simulink model "ASM_Traffic_MultiCore"  (R2026a)
settings: Solver=ode1  StartTime=SIM.tstart.v  StopTime=SIM.tend.v  FixedStep=SIM.StepSize.v
PostLoadFcn:
  | if any(exist('dsrtsu_mdlpostloadfcn', 'file') ~= 0), dsrtsu_mdlpostloadfcn('Execute', bdroot); end
  | try, asm_mdl_postloadfcn(bdroot, 'UpdateModel', 3600); catch, disp(lasterr); end,
InitFcn:
  | , if any(exist('rtifpga_mdlclblib', 'file') ~= 0), rtifpga_mdlclblib('Init', bdroot); end,
  | , if any(exist('dsmpb_private', 'file') ~= 0), dsmpb_private('dsmpb_mdlclblib', 'Init', bdroot); end,
model workspace (MAT data in the model file):
  asmReferencePath = [0 0.01 0.02 0.03 0.04 0.05 0.06 0.07 0.08 0.09 0.1 0.11 ... (350007 elements, 50001x7)]
  roadBounds : Simulink.Parameter (value not decoded)
  safetyAxes : Simulink.Parameter (value not decoded)
undefined symbols (not defined in the file): _to_, a0b2, ASM_BrakeHydraulics_DemoSystems, ASM_VehicleDynamics_DemoSystems, b98103fe8ad365046cd0, BrakeCircuit, controllerConfig, CPT, Crankshaft, DiscIntNeverNeededParam, dsmsi, FinalDriveAssembly, MDL, ModeSignals, mu, Pos_BrakePedal_Maneuver, rad, RefSignals, roadFamilyData, roadFamilyId, s_to_rpm, SIM, SoftECU, Suspension, Tire, Transmission
libraries: ASM_Traffic_lib x135, simulink x98, ASM_Utils_lib x77, ASM_VehicleDynamics_lib x70, ASM_Environment_lib x22, dsmpblib x20, dsmsilib x15, MDLD_Utils_lib x10, ASM_BrakeHydraulics_lib x3, sl_discontinuities x2
(part 37 of 65)

== system ASM_Traffic_MultiCore/Driver/Plant/Driver/ReferenceVelocity/Reduce_Dimension2 ==
  In : Inport
  Selector : Selector  InputPortWidth=15  IndexOptions=Index vector (dialog)  Indices=[8:10]  OutputSizes=1
      settings: AttributesFormatString=|
      | PortWidth = %<InputPortWidth>
      | Indices = %<Indices>
  UnitConversion2 : ASM_Utils_lib/UnitConversion/UnitConversion  Selection=km/h_to_m/s
  Out : Outport  VectorParamsAs1DForOutWhenUnconnected=off
  wires:
  UnitConversion2/1 -> Selector/1
  In/1 -> UnitConversion2/1
  Selector/1 -> Out/1

== system ASM_Traffic_MultiCore/Driver/Plant/Driver/ReferenceVelocity/Reduce_Dimension3 ==
  In : Inport
  Selector : Selector  InputPortWidth=15  IndexOptions=Index vector (dialog)  Indices=[1:10]  OutputSizes=1
      settings: AttributesFormatString=|
      | PortWidth = %<InputPortWidth>
      | Indices = %<Indices>
  Out : Outport  VectorParamsAs1DForOutWhenUnconnected=off
  wires:
  In/1 -> Selector/1
  Selector/1 -> Out/1

== system ASM_Traffic_MultiCore/Driver/Plant/Driver/ReferenceVelocity/Reduce_Dimension4 ==
  In : Inport
  Selector : Selector  InputPortWidth=10  IndexOptions=Index vector (dialog)  Indices=[8:10]  OutputSizes=1
      settings: AttributesFormatString=|
      | PortWidth = %<InputPortWidth>
      | Indices = %<Indices>
  Out : Outport  VectorParamsAs1DForOutWhenUnconnected=off
  wires:
  Selector/1 -> Out/1
  In/1 -> Selector/1

== system ASM_Traffic_MultiCore/Driver/Plant/UserInterface/DISP_Plant/Angle_SteeringWheel[deg] ==
  In1 : Inport
  Out1 : Outport  VectorParamsAs1DForOutWhenUnconnected=off
  wires:
  In1/1 -> Out1/1

== system ASM_Traffic_MultiCore/Driver/Plant/UserInterface/DISP_Plant/Err ==
  Current : Inport
  Set : Inport  Port=2
  Sum : Sum  Inputs=|+-  InputSameDT=on  SaturateOnIntegerOverflow=on  OutDataTypeStr=Inherit: Same as first input
  Error[km|h] : Outport  VectorParamsAs1DForOutWhenUnconnected=off
  wires:
  Current/1 -> Sum/1
  Set/1 -> Sum/2
  Sum/1 -> Error[km|h]/1

== system ASM_Traffic_MultiCore/Driver/Plant/UserInterface/DISP_Plant/Gear[] ==
  In1 : Inport
  Out1 : Outport  VectorParamsAs1DForOutWhenUnconnected=off
  wires:
  In1/1 -> Out1/1

== system ASM_Traffic_MultiCore/Driver/Plant/UserInterface/DISP_Plant/Pos_AccPedal[%] ==
  In1 : Inport
  Out1 : Outport  VectorParamsAs1DForOutWhenUnconnected=off
  wires:
  In1/1 -> Out1/1

== system ASM_Traffic_MultiCore/Driver/Plant/UserInterface/DISP_Plant/Pos_BrakePedal[%] ==
  In1 : Inport
  Out1 : Outport  VectorParamsAs1DForOutWhenUnconnected=off
  wires:
  In1/1 -> Out1/1

== system ASM_Traffic_MultiCore/Driver/Plant/UserInterface/DISP_Plant/Pos_ClutchPedal[%] ==
  In1 : Inport
  Out1 : Outport  VectorParamsAs1DForOutWhenUnconnected=off
  wires:
  In1/1 -> Out1/1

== system ASM_Traffic_MultiCore/Driver/Plant/UserInterface/DISP_Plant/RelativeErr ==
  Current : Inport
  Set : Inport  Port=2
  AvoidNAN : Fcn  Expr=u/(u*u+1.E-20)
  Limit_RelativeError : Saturate  UpperLimit=UpLim  LowerLimit=LowLim
  Product : Product  InputSameDT=on  SaturateOnIntegerOverflow=on  OutDataTypeStr=Inherit: Same as first input
  Sum : Sum  Inputs=|+-  InputSameDT=on  SaturateOnIntegerOverflow=on  OutDataTypeStr=Inherit: Same as first input
  "[0_1]2[%]" : Gain  Gain=100  SaturateOnIntegerOverflow=on  OutDataTypeStr=Inherit: Same as input  ParamDataTypeStr=Inherit: Same as input
  RelativeError[%] : Outport  VectorParamsAs1DForOutWhenUnconnected=off
  wires:
  AvoidNAN/1 -> Product/2
  Current/1 -> Sum/1
  Product/1 -> "[0_1]2[%]"/1
  Set/1 -> AvoidNAN/1, Sum/2
  Sum/1 -> Product/1
  "[0_1]2[%]"/1 -> Limit_RelativeError/1
  Limit_RelativeError/1 -> RelativeError[%]/1

== system ASM_Traffic_MultiCore/Driver/Plant/UserInterface/DISP_Plant/SelectorLever[-3T|-2P|-1R|0N|1D] ==
  In1 : Inport
  Out1 : Outport  VectorParamsAs1DForOutWhenUnconnected=off
  wires:
  In1/1 -> Out1/1

== system ASM_Traffic_MultiCore/Driver/Plant/UserInterface/DISP_Plant/a_x_Vehicle_Ref[m|s2] ==
  In1 : Inport
  Out1 : Outport  VectorParamsAs1DForOutWhenUnconnected=off
  wires:
  In1/1 -> Out1/1

== system ASM_Traffic_MultiCore/Driver/Plant/UserInterface/DISP_Plant/e_Lat[m] ==
  In1 : Inport
  Out1 : Outport  VectorParamsAs1DForOutWhenUnconnected=off
  wires:
  In1/1 -> Out1/1

== system ASM_Traffic_MultiCore/Driver/Plant/UserInterface/DISP_Plant/v_Vehicle[km|h] ==
  In1 : Inport
  Out1 : Outport  VectorParamsAs1DForOutWhenUnconnected=off
  wires:
  In1/1 -> Out1/1

== system ASM_Traffic_MultiCore/Driver/Plant/UserInterface/DISP_Plant/v_Vehicle_Ref[km|h] ==
  In1 : Inport
  Out1 : Outport  VectorParamsAs1DForOutWhenUnconnected=off
  wires:
  In1/1 -> Out1/1

== system ASM_Traffic_MultiCore/Driver/SignalInterface/ASMSignalInterface/signal_structure/InfoBlock ==

== system ASM_Traffic_MultiCore/Drivetrain/Control/SoftECU_Drivetrain/SoftECU_Transmission/ASMSignalCollector ==
  BusCreator : BusCreator  Inputs=5
  ASMSignalBus : Outport  VectorParamsAs1DForOutWhenUnconnected=off
  wires:
  BusCreator/1 -> ASMSignalBus/1  "Control"
  [ASMBUS_SOFTECU_LOCKUP_CLUTCH_CONTROL] -> BusCreator/1
  [ASMBUS_SOFTECU_SHIFT_LOCK_CONTROL] -> BusCreator/2
  [ASMBUS_SOFTECU_SHIFT_STRATEGY] -> BusCreator/3
  [ASMBUS_SOFTECU_TIP_SHIFT_CONTROL] -> BusCreator/4
  [ASMBUS_SOFTECU_TORQUE_INTERVENTION_CONTROL] -> BusCreator/5

== system ASM_Traffic_MultiCore/Drivetrain/Control/SoftECU_Drivetrain/SoftECU_Transmission/SOFTECU_SETUP ==
  Gear_Max_Maneuver[0Off|1_n] : Inport
  SOFTECU_TRANSMISSION_SETUP : ASM_VehicleDynamics_lib/SoftECU/SoftECU_Transmission/SOFTECU_TRANSMISSION_SETUP  Tag=ASM_SUBCOMPONENT  Const_Max_num_Gear=MDL.SoftECU.SoftECUTransmission.Const_Max_num_Gear  ASMProperties=struct('Name','SOFTECU_TRANSMISSION_SETUP','Version','1.0','Library','ASM_VehicleDynamics_lib')  ASMInstanceName=softecu_transmission_setup  ASMInstanceID=1
  Terminator : Terminator
  tag scope: TAG_SoftECU_Const_Max_num_Gear=scoped
  wires:
  SOFTECU_TRANSMISSION_SETUP/1 -> [TAG_SoftECU_Const_Max_num_Gear]
  [TAG_SoftECU_Const_Max_num_Gear] -> Terminator/1
  Gear_Max_Maneuver[0Off|1_n]/1 -> SOFTECU_TRANSMISSION_SETUP/1

== system ASM_Traffic_MultiCore/Drivetrain/Control/SoftECU_Drivetrain/SoftECU_Transmission/State_Engine ==
  note: Consider the engine to be active, if StartStop system is active
  In[] : Inport
  State_StartStop[1Off|2NotReady|3Ready|4EngStopped] : Inport  Port=2
  Data Type Conversion : DataTypeConversion  OutDataTypeStr=double  SaturateOnIntegerOverflow=off  RndMeth=Floor
  Engine_Active : Constant  Value=3
  NotOff : simulink/Logic and Bit Operations/Compare To Constant  relop=~=  const=1  OutDataTypeStr=boolean
  Switch : Switch  Criteria=u2 ~= 0  SaturateOnIntegerOverflow=off  InputSameDT=off
  Out[] : Outport  VectorParamsAs1DForOutWhenUnconnected=off
  wires:
  State_StartStop[1Off|2NotReady|3Ready|4EngStopped]/1 -> NotOff/1
  Data Type Conversion/1 -> Switch/3
  NotOff/1 -> Switch/2
  Switch/1 -> Out[]/1
  Engine_Active/1 -> Switch/1
  In[]/1 -> Data Type Conversion/1

== system ASM_Traffic_MultiCore/Drivetrain/Control/SoftECU_Drivetrain/SoftECU_Transmission/Sw_Gear ==
  In[] : Inport
  Ext : Constant
  OR : Logic  Operator=OR  AllPortsSameDT=off  OutDataTypeStr=boolean
  Ref : simulink/Logic and Bit Operations/Compare To Constant  relop===  const=4  OutDataTypeStr=boolean
  SoftECU : Constant  Value=2
  Stim : simulink/Logic and Bit Operations/Compare To Constant  relop===  const=1  OutDataTypeStr=boolean
  Switch : Switch  Criteria=u2 ~= 0  SaturateOnIntegerOverflow=off  InputSameDT=off
  Terminator : Terminator
  Out[] : Outport  VectorParamsAs1DForOutWhenUnconnected=off
  wires:
  Switch/1 -> Terminator/1
  SoftECU/1 -> Switch/3, Out[]/1
  Ext/1 -> Switch/1
  OR/1 -> Switch/2
  Ref/1 -> OR/2
  Stim/1 -> OR/1
  In[]/1 -> Ref/1, Stim/1

== system ASM_Traffic_MultiCore/Drivetrain/Control/SoftECU_Drivetrain/SoftECU_Transmission/Sw_LockupClutch ==
  In[] : Inport
  SoftECU : Constant  Value=2
  Terminator : Terminator
  Out[] : Outport  VectorParamsAs1DForOutWhenUnconnected=off
  wires:
  SoftECU/1 -> Out[]/1
  In[]/1 -> Terminator/1

== system ASM_Traffic_MultiCore/Drivetrain/Control/SoftECU_Drivetrain/SoftECU_Transmission/Unit Delay ==
  In1 : Inport
  Reset_States[0|1] : Inport  Port=2
  Unit Delay Resettable1 : Delay  DelayLength=1  InitialCondition=0  ExternalReset=Level
      settings: InputPortMap=u0,r5
  Out1 : Outport  VectorParamsAs1DForOutWhenUnconnected=off
  wires:
  Reset_States[0|1]/1 -> Unit Delay Resettable1/2
  In1/1 -> Unit Delay Resettable1/1
  Unit Delay Resettable1/1 -> Out1/1

== system ASM_Traffic_MultiCore/Drivetrain/Control/SoftECU_Drivetrain/SoftECU_Transmission/Unit Delay2 ==
  In1 : Inport
  Reset_States[0|1] : Inport  Port=2
  Unit Delay Resettable1 : Delay  DelayLength=1  InitialCondition=100  ExternalReset=Level
      settings: InputPortMap=u0,r5
  Out1 : Outport  VectorParamsAs1DForOutWhenUnconnected=off
  wires:
  Reset_States[0|1]/1 -> Unit Delay Resettable1/2
  In1/1 -> Unit Delay Resettable1/1
  Unit Delay Resettable1/1 -> Out1/1

== system ASM_Traffic_MultiCore/Drivetrain/Control/UserInterface/DISP_Control/Ctrl_Lockup_Clutch[0_1] ==
  In1 : Inport
  Out1 : Outport  VectorParamsAs1DForOutWhenUnconnected=off
  wires:
  In1/1 -> Out1/1

== system ASM_Traffic_MultiCore/Drivetrain/Control/UserInterface/DISP_Control/Ctrl_Parking_Pawl[0|1] ==
  In1 : Inport
  Out1 : Outport  VectorParamsAs1DForOutWhenUnconnected=off
  wires:
  In1/1 -> Out1/1

== system ASM_Traffic_MultiCore/Drivetrain/Control/UserInterface/DISP_Control/Factor_Trq_Engine_Red[%] ==
  In1 : Inport
  Out1 : Outport  VectorParamsAs1DForOutWhenUnconnected=off
  wires:
  In1/1 -> Out1/1

== system ASM_Traffic_MultiCore/Drivetrain/Control/UserInterface/DISP_Control/Gear[] ==
  In1 : Inport
  Out1 : Outport  VectorParamsAs1DForOutWhenUnconnected=off
  wires:
  In1/1 -> Out1/1

== system ASM_Traffic_MultiCore/Drivetrain/Plant/Drivetrain/Final_Drive_Assembly/ASMSignalCollector ==
  Bus Selector1 : BusSelector  OutputSignals=Shaft_FL,Shaft_FR
  Bus Selector2 : BusSelector  OutputSignals=Shaft_RL,Shaft_RR
  BusCreator : BusCreator  Inputs=18
  Clutch_4WD : Subsystem
  Dummy_TGCL4WD_Shaft : Subsystem
  FinalDriveRatio : Subsystem
  Shaft_CF : Subsystem
  Shaft_CR : Subsystem
  Transfer_Gearbox : Subsystem
  Trq_Shafts : Subsystem
  tag scope: ASMBUS_Drivetrain_FinalDriveAssembly=scoped
  wires:
  Trq_Shafts/2(Trq_Shaft[FL;FR;RL;RR][Nm]) -> BusCreator/18
  Trq_Shafts/1(Trq_Out_Front_Diff[Nm]) -> BusCreator/17
  FinalDriveRatio/4(i_FinalDrive[]) -> BusCreator/4
  FinalDriveRatio/3(TrqDistri_Front_Rear[0_1]) -> BusCreator/3
  FinalDriveRatio/2(i_RearDrive[]) -> BusCreator/2
  FinalDriveRatio/1(i_FrontDrive[]) -> BusCreator/1
  BusCreator/1 -> [ASMBUS_Drivetrain_FinalDriveAssembly]  "FinalDriveAssembly"
  Bus Selector2/2 -> BusCreator/16, Trq_Shafts/4(Shaft_RR)  "<Shaft_RR>"
  Bus Selector2/1 -> BusCreator/15, Trq_Shafts/3(Shaft_RL)  "<Shaft_RL>"
  Bus Selector1/2 -> BusCreator/14, Trq_Shafts/2(Shaft_FR)  "<Shaft_FR>"
  Bus Selector1/1 -> BusCreator/13, Trq_Shafts/1(Shaft_FL)  "<Shaft_FL>"
  Clutch_4WD/1(ASMSignalBus) -> BusCreator/12
  Transfer_Gearbox/1(ASMSignalBus) -> BusCreator/11
  [ASMBUS_Drivetrain_CentralDifferential] -> FinalDriveRatio/2(CentralDifferential), BusCreator/5
  Dummy_TGCL4WD_Shaft/1(Out) -> BusCreator/8
  [ASMBUS_Drivetrain_RearDifferential] -> BusCreator/7, FinalDriveRatio/4(RearDifferential), Bus Selector2/1
  [ASMBUS_Drivetrain_FrontDifferential] -> BusCreator/6, FinalDriveRatio/3(FrontDifferential), Bus Selector1/1
  Shaft_CF/1(ASMSignalBus) -> BusCreator/9
  Shaft_CR/1(ASMSignalBus) -> BusCreator/10
  [ASMBUS_Drivetrain_Mode] -> Shaft_CF/1(Mode_Drivetrain[1|2|3|4|5]), Clutch_4WD/1(Mode_Drivetrain[1|2|3|4|5]), Transfer_Gearbox/1(Mode_Drivetrain[1|2|3|4|5]), Shaft_CR/1(Mode_Drivetrain[1|2|3|4|5]), FinalDriveRatio/1(Drivetrain_Mode[1|2|3|4|5])

== system ASM_Traffic_MultiCore/Drivetrain/Plant/Drivetrain/Final_Drive_Assembly/Differentials ==
  omega_Wheel[FL,FR,RL,RR][rad|s] : Inport
  Trq_Out_Trm[Nm] : Inport  Port=2
  Trq_In_FrontDiff[Nm] : Inport  Port=3
  Trq_In_RearDiff[Nm] : Inport  Port=4
  drive_trq[Nm] : Inport  Port=5
  Bus Selector1 : BusSelector  OutputSignals=Ctrl_FrontDiff[0_1]
  Bus Selector2 : BusSelector  OutputSignals=Ctrl_CentralDiff[0_1]
  Bus Selector4 : BusSelector  OutputSignals=Ctrl_RearDiff[0_1]
  CENTRAL_DIFFERENTIAL_RIGID : ASM_VehicleDynamics_lib/Drivetrain/Differential/CENTRAL_DIFFERENTIAL_RIGID  Tag=ASM_SUBCOMPONENT  Const_TrqDistribution=MDL.Drivetrain.CentralDifferentialRigid.Const_TrqDistribution  Const_i_MainReductionGear=MDL.Drivetrain.CentralDifferentialRigid.Const_i_MainReductionGear  Const_Trq_Max_LockClutch=MDL.Drivetrain.CentralDifferentialRigid.Const_Trq_Max_LockClutch  Const_Ctrl_Offset_LockClutch=MDL.Drivetrain.CentralDifferentialRigid.Const_Ctrl_Offset_LockClutch  Const_Stiffness_Fric_CentralDiff=MDL.Drivetrain.CentralDifferentialRigid.Const_Stiffness_Fric_CentralDiff  Const_Damping_Fric_CentralDiff=MDL.Drivetrain.CentralDifferentialRigid.Const_Damping_Fric_CentralDiff  StepSize=SIM.StepSize  ASMProperties=struct('Name','CENTRAL_DIFFERENTIAL_RIGID','Version','3.0','Library','ASM_VehicleDynamics_lib')  ASMInstanceName=central_differential_rigid  ASMInstanceID=1
  FRONT_DIFFERENTIAL_RIGID : ASM_VehicleDynamics_lib/Drivetrain/Differential/FRONT_DIFFERENTIAL_RIGID  Tag=ASM_SUBCOMPONENT  Const_i_MainReductionGear=MDL.Drivetrain.FrontDifferentialRigid.Const_i_MainReductionGear  Const_Trq_Max_LockClutch=MDL.Drivetrain.FrontDifferentialRigid.Const_Trq_Max_LockClutch  Const_Ctrl_Offset_LockClutch=MDL.Drivetrain.FrontDifferentialRigid.Const_Ctrl_Offset_LockClutch  Const_Stiffness_Fric_FrontDiff=MDL.Drivetrain.FrontDifferentialRigid.Const_Stiffness_Fric_FrontDiff  Const_Damping_Fric_FrontDiff=MDL.Drivetrain.FrontDifferentialRigid.Const_Damping_Fric_FrontDiff  StepSize=SIM.StepSize  ASMProperties=struct('Name','FRONT_DIFFERENTIAL_RIGID','Version','4.0','Library','ASM_VehicleDynamics_lib')  ASMInstanceName=front_differential_rigid  ASMInstanceID=1
  Map_Mode_2_Parameter : Lookup_n-D  NumberOfTableDimensions=1  BreakpointsForDimension1=[1:5]  Table=[1 2 3 1 2]  InternalRulePriority=Speed  RndMeth=Simplest
      settings: AttributesFormatString=Map FF => FWD & FF4WD => AWD
  Mux : Mux
  REAR_DIFFERENTIAL_RIGID : ASM_VehicleDynamics_lib/Drivetrain/Differential/REAR_DIFFERENTIAL_RIGID  Tag=ASM_SUBCOMPONENT  Const_i_MainReductionGear=MDL.Drivetrain.RearDifferentialRigid.Const_i_MainReductionGear  Const_Trq_Max_LockClutch=MDL.Drivetrain.RearDifferentialRigid.Const_Trq_Max_LockClutch  Const_Ctrl_Offset_LockClutch=MDL.Drivetrain.RearDifferentialRigid.Const_Ctrl_Offset_LockClutch  Const_Stiffness_Fric_RearDiff=MDL.Drivetrain.RearDifferentialRigid.Const_Stiffness_Fric_RearDiff  Const_Damping_Fric_RearDiff=MDL.Drivetrain.RearDifferentialRigid.Const_Damping_Fric_RearDiff  StepSize=SIM.StepSize  ASMProperties=struct('Name','REAR_DIFFERENTIAL_RIGID','Version','4.0','Library','ASM_VehicleDynamics_lib')  ASMInstanceName=rear_differential_rigid  ASMInstanceID=1
  Saturation[1_3] : Saturate  UpperLimit=3  LowerLimit=1
  SignalSelection : Subsystem
  Sw_Axle_Driven_FrontDiff : Subsystem
  Sw_Axle_Driven_RearDiff : Subsystem
  Switch_Trq_shaft : Switch  Criteria=u2 ~= 0  SaturateOnIntegerOverflow=off  InputSameDT=off
  Trq_shaft_switch : Constant  Value=0
  UnitConversion : ASM_Utils_lib/UnitConversion/UnitConversion  Selection=[0_1]_to_%
  UnitConversion1 : ASM_Utils_lib/UnitConversion/UnitConversion  Selection=[0_1]_to_%
  UnitConversion2 : ASM_Utils_lib/UnitConversion/UnitConversion  Selection=[0_1]_to_%
  avoid_incomplete_trace2source : Subsystem
  avoid_incomplete_trace2source1 : Subsystem
  omega_Cage_CentralDiff[rad|s] : Terminator
  omega_Cage_RearDiff[rad|s] : Terminator
  omega_Wheel[FL][rad|s] : Selector  InputPortWidth=4  IndexOptions=Index vector (dialog)  Indices=[1]  OutputSizes=1
  omega_Wheel[FR][rad|s] : Selector  InputPortWidth=4  IndexOptions=Index vector (dialog)  Indices=[2]  OutputSizes=1
  omega_Wheel[RL][rad|s] : Selector  InputPortWidth=4  IndexOptions=Index vector (dialog)  Indices=[3]  OutputSizes=1
  omega_Wheel[RR][rad|s] : Selector  InputPortWidth=4  IndexOptions=Index vector (dialog)  Indices=[4]  OutputSizes=1
  omega_In_Diff[rad|s] : Outport  VectorParamsAs1DForOutWhenUnconnected=off
  Trq_Shaft[FL,FR,RL,RR][Nm] : Outport  Port=2  VectorParamsAs1DForOutWhenUnconnected=off
  omega_Cage_FrontDiff[rad|s] : Outport  Port=3  VectorParamsAs1DForOutWhenUnconnected=off
  omega_In_RearDiff[rad|s] : Outport  Port=4  VectorParamsAs1DForOutWhenUnconnected=off
  Trq_Out_Front_CentralDiff[Nm] : Outport  Port=5  VectorParamsAs1DForOutWhenUnconnected=off
  Trq_Out_Rear_CentralDiff[Nm] : Outport  Port=6  VectorParamsAs1DForOutWhenUnconnected=off
  tag scope: ASMBUS_Drivetrain_CentralDifferential=scoped, ASMBUS_Drivetrain_FrontDifferential=scoped, ASMBUS_Drivetrain_RearDifferential=scoped
  wires:
  avoid_incomplete_trace2source1/1(Out1) -> CENTRAL_DIFFERENTIAL_RIGID/6
  avoid_incomplete_trace2source/1(Out1) -> CENTRAL_DIFFERENTIAL_RIGID/5
  omega_Wheel[FL,FR,RL,RR][rad|s]/1 -> omega_Wheel[RR][rad|s]/1, omega_Wheel[RL][rad|s]/1, omega_Wheel[FR][rad|s]/1, omega_Wheel[FL][rad|s]/1
  omega_Wheel[RR][rad|s]/1 -> REAR_DIFFERENTIAL_RIGID/6
  omega_Wheel[RL][rad|s]/1 -> REAR_DIFFERENTIAL_RIGID/5
  omega_Wheel[FR][rad|s]/1 -> FRONT_DIFFERENTIAL_RIGID/6
  omega_Wheel[FL][rad|s]/1 -> FRONT_DIFFERENTIAL_RIGID/5
  UnitConversion2/1 -> REAR_DIFFERENTIAL_RIGID/4
  UnitConversion1/1 -> FRONT_DIFFERENTIAL_RIGID/4
  UnitConversion/1 -> CENTRAL_DIFFERENTIAL_RIGID/4
  [ASMBUS_Drivetrain_ECU_Signals] -> Bus Selector2/1, Bus Selector1/1, Bus Selector4/1
  Sw_Axle_Driven_RearDiff/1(Out[]) -> REAR_DIFFERENTIAL_RIGID/1
  Sw_Axle_Driven_FrontDiff/1(Out[]) -> FRONT_DIFFERENTIAL_RIGID/1
  Map_Mode_2_Parameter/1 -> Saturation[1_3]/1
  Trq_In_RearDiff[Nm]/1 -> REAR_DIFFERENTIAL_RIGID/3
  Trq_In_FrontDiff[Nm]/1 -> FRONT_DIFFERENTIAL_RIGID/3
  CENTRAL_DIFFERENTIAL_RIGID/5 -> Trq_Out_Rear_CentralDiff[Nm]/1
  CENTRAL_DIFFERENTIAL_RIGID/4 -> Trq_Out_Front_CentralDiff[Nm]/1
  REAR_DIFFERENTIAL_RIGID/2 -> avoid_incomplete_trace2source/1(In1), omega_In_RearDiff[rad|s]/1
  REAR_DIFFERENTIAL_RIGID/3 -> omega_Cage_RearDiff[rad|s]/1
  REAR_DIFFERENTIAL_RIGID/5 -> Mux/4
  REAR_DIFFERENTIAL_RIGID/4 -> Mux/3
  FRONT_DIFFERENTIAL_RIGID/5 -> Mux/2
  FRONT_DIFFERENTIAL_RIGID/4 -> Mux/1
  Mux/1 -> Switch_Trq_shaft/1
  FRONT_DIFFERENTIAL_RIGID/3 -> omega_Cage_FrontDiff[rad|s]/1
  CENTRAL_DIFFERENTIAL_RIGID/3 -> omega_Cage_CentralDiff[rad|s]/1
  Trq_Out_Trm[Nm]/1 -> CENTRAL_DIFFERENTIAL_RIGID/3
  CENTRAL_DIFFERENTIAL_RIGID/1 -> [ASMBUS_Drivetrain_CentralDifferential]
  REAR_DIFFERENTIAL_RIGID/1 -> [ASMBUS_Drivetrain_RearDifferential]
  Bus Selector4/1 -> UnitConversion2/1  "<Ctrl_RearDiff[0_1]>"
  Bus Selector1/1 -> UnitConversion1/1  "<Ctrl_FrontDiff[0_1]>"
  Bus Selector2/1 -> UnitConversion/1  "<Ctrl_CentralDiff[0_1]>"
  FRONT_DIFFERENTIAL_RIGID/2 -> avoid_incomplete_trace2source1/1(In1), SignalSelection/2(omega_In_FrontDiff[rad|s])
  SignalSelection/1(omega_In_Diff[rad|s]) -> omega_In_Diff[rad|s]/1
  [ASMBUS_Drivetrain_Mode] -> Map_Mode_2_Parameter/1
  Saturation[1_3]/1 -> Sw_Axle_Driven_RearDiff/1(In[]), Sw_Axle_Driven_FrontDiff/1(In[]), CENTRAL_DIFFERENTIAL_RIGID/1
  [ASMBUS_Drivetrain_Reset] -> REAR_DIFFERENTIAL_RIGID/2, FRONT_DIFFERENTIAL_RIGID/2, CENTRAL_DIFFERENTIAL_RIGID/2
  CENTRAL_DIFFERENTIAL_RIGID/2 -> SignalSelection/1(omega_In_CentralDiff[rad|s])
  FRONT_DIFFERENTIAL_RIGID/1 -> [ASMBUS_Drivetrain_FrontDifferential]
  Switch_Trq_shaft/1 -> Trq_Shaft[FL,FR,RL,RR][Nm]/1
  Trq_shaft_switch/1 -> Switch_Trq_shaft/2
  drive_trq[Nm]/1 -> Switch_Trq_shaft/3

== system ASM_Traffic_MultiCore/Drivetrain/Plant/Drivetrain/Final_Drive_Assembly/FF4WD_Parts ==
  omega_In_RearDiff[rad|s] : Inport
  omega_Cage_FrontDiff[rad|s] : Inport  Port=2
  Bus Selector4 : BusSelector  OutputSignals=Ctrl_Clutch_4WD[0_1]
  CLUTCH_4WD_RIGID : ASM_VehicleDynamics_lib/Drivetrain/Clutch/CLUTCH_4WD_RIGID  Tag=ASM_SUBCOMPONENT  Const_Torque_Max=MDL.Drivetrain.Clutch4WDRigid.Const_Torque_Max  Map_Trq_Clutch_Red=MDL.Drivetrain.Clutch4WDRigid.Map_Trq_Clutch_Red  Const_Stiffness_Fric_Clutch_4WD=MDL.Drivetrain.Clutch4WDRigid.Const_Stiffness_Fric_Clutch_4WD  Const_Damping_Fric_Clutch_4WD=MDL.Drivetrain.Clutch4WDRigid.Const_Damping_Fric_Clutch_4WD  StepSize=SIM.StepSize  ASMProperties=struct('Name','CLUTCH_4WD_RIGID','Version','2.0','Library','ASM_VehicleDynamics_lib')  ASMInstanceName=clutch_4wd_rigid  ASMInstanceID=1
  TRANSFER_GEARBOX_RIGID : ASM_VehicleDynamics_lib/Drivetrain/Gearbox/TRANSFER_GEARBOX_RIGID  Tag=ASM_SUBCOMPONENT  Const_GearRatio=MDL.Drivetrain.TransferGearboxRigid.Const_GearRatio  ASMProperties=struct('Name','TRANSFER_GEARBOX_RIGID','Version','1.0','Library','ASM_VehicleDynamics_lib')  ASMInstanceName=transfer_gearbox_rigid  ASMInstanceID=1
  UnitConversion : ASM_Utils_lib/UnitConversion/UnitConversion  Selection=[0_1]_to_%
  avoid_incomplete_trace2source : Subsystem
  avoid_incomplete_trace2source1 : Subsystem
  Trq_Lock_Clutch4WD[Nm] : Outport  VectorParamsAs1DForOutWhenUnconnected=off
  tag scope: ASMBUS_Drivetrain_Clutch_4WD=scoped, ASMBUS_Drivetrain_Transfer_Gearbox=scoped
  wires:
  avoid_incomplete_trace2source1/1(Out1) -> CLUTCH_4WD_RIGID/4
  omega_In_RearDiff[rad|s]/1 -> avoid_incomplete_trace2source1/1(In1)
  avoid_incomplete_trace2source/1(Out1) -> CLUTCH_4WD_RIGID/1
  TRANSFER_GEARBOX_RIGID/2 -> avoid_incomplete_trace2source/1(In1)
  [ASMBUS_Drivetrain_ECU_Signals] -> Bus Selector4/1
  UnitConversion/1 -> CLUTCH_4WD_RIGID/2
  TRANSFER_GEARBOX_RIGID/1 -> [ASMBUS_Drivetrain_Transfer_Gearbox]
  omega_Cage_FrontDiff[rad|s]/1 -> TRANSFER_GEARBOX_RIGID/1
  CLUTCH_4WD_RIGID/2 -> Trq_Lock_Clutch4WD[Nm]/1
  [ASMBUS_Drivetrain_Reset] -> CLUTCH_4WD_RIGID/3
  CLUTCH_4WD_RIGID/1 -> [ASMBUS_Drivetrain_Clutch_4WD]
  Bus Selector4/1 -> UnitConversion/1  "<Ctrl_Clutch_4WD[0_1]>"

== system ASM_Traffic_MultiCore/Drivetrain/Plant/Drivetrain/Final_Drive_Assembly/SignalSelection ==
  Trq_Out_Trm[Nm] : Inport
  Trq_Lock_Clutch4WD[Nm] : Inport  Port=2
  Trq_Out_Front_CentralDiff[Nm] : Inport  Port=3
  Trq_Out_Rear_CentralDiff[Nm] : Inport  Port=4
  AWD : simulink/Logic and Bit Operations/Compare To Constant  relop===  const=1  OutDataTypeStr=boolean
  FWD : simulink/Logic and Bit Operations/Compare To Constant  relop===  const=2  OutDataTypeStr=boolean
  OR : Logic  Operator=OR  Inputs=3  AllPortsSameDT=off  OutDataTypeStr=boolean
  RWD : simulink/Logic and Bit Operations/Compare To Constant  relop===  const=3  OutDataTypeStr=boolean
  Saturation[1_5] : Saturate  UpperLimit=5  LowerLimit=1
  Switch : Switch  Criteria=u2 ~= 0  SaturateOnIntegerOverflow=off  InputSameDT=off
  Switch1 : Switch  Criteria=u2 ~= 0  SaturateOnIntegerOverflow=off  InputSameDT=off
  Trq_In_FrontDiff[Nm] : Outport  VectorParamsAs1DForOutWhenUnconnected=off
  Trq_In_RearDiff[Nm] : Outport  Port=2  VectorParamsAs1DForOutWhenUnconnected=off
  wires:
  Trq_Lock_Clutch4WD[Nm]/1 -> Switch1/3
  Trq_Out_Rear_CentralDiff[Nm]/1 -> Switch1/1
  Switch1/1 -> Trq_In_RearDiff[Nm]/1
  Switch/1 -> Trq_In_FrontDiff[Nm]/1
  Trq_Out_Trm[Nm]/1 -> Switch/3
  OR/1 -> Switch/2, Switch1/2
  Trq_Out_Front_CentralDiff[Nm]/1 -> Switch/1
  AWD/1 -> OR/1
  FWD/1 -> OR/2
  RWD/1 -> OR/3
  Saturation[1_5]/1 -> RWD/1, FWD/1, AWD/1
  [ASMBUS_Drivetrain_Mode] -> Saturation[1_5]/1

== system ASM_Traffic_MultiCore/Drivetrain/Plant/Drivetrain/Transmission/ASMSignalCollector ==
  Mode_Transmission[1|2] : Inport
  Gear_MT[] : Inport  Port=2
  Gear_AT[] : Inport  Port=3
  Bus Selector : BusSelector  OutputSignals=i_unsync_Trm[],i_Trm[],Trq_Out_Trm[Nm],omega_In_Trm[rad|s],Inertia_Trm[kgm2],omega_Out_Trm[rad|s]
  Bus Selector1 : BusSelector  OutputSignals=GearBox
  Bus Selector3 : BusSelector  OutputSignals=GearBox
  BusCreator : BusCreator  Inputs=3
  BusCreator1 : BusCreator  Inputs=7
  Multiport Switch1 : MultiPortSwitch  Inputs=2  InputSameDT=off
  Multiport Switch3 : MultiPortSwitch  Inputs=2  InputSameDT=off
  tag scope: ASMBUS_Drivetrain_Transmission=scoped
  wires:
  Mode_Transmission[1|2]/1 -> Multiport Switch1/1, Multiport Switch3/1
  BusCreator/1 -> [ASMBUS_Drivetrain_Transmission]  "Transmission"
  [ASMBUS_ManualTransmission] -> Bus Selector3/1, BusCreator/1
  [ASMBUS_AutomaticTransmission] -> Bus Selector1/1, BusCreator/2
  BusCreator1/1 -> BusCreator/3  "OutputSignals"
  Multiport Switch3/1 -> Bus Selector/1
  Multiport Switch1/1 -> BusCreator1/7  "Gear[]"
  Bus Selector3/1 -> Multiport Switch3/2  "<GearBox>"
  Bus Selector1/1 -> Multiport Switch3/3  "<GearBox>"
  Bus Selector/1 -> BusCreator1/1  "<i_unsync_Trm[]>"
  Bus Selector/2 -> BusCreator1/2  "<i_Trm[]>"
  Bus Selector/3 -> BusCreator1/3  "<Trq_Out_Trm[Nm]>"
  Bus Selector/4 -> BusCreator1/4  "<omega_In_Trm[rad|s]>"
  Bus Selector/5 -> BusCreator1/5  "<Inertia_Trm[kgm2]>"
  Bus Selector/6 -> BusCreator1/6  "<omega_Out_Trm[rad|s]>"
  Gear_MT[]/1 -> Multiport Switch1/2
  Gear_AT[]/1 -> Multiport Switch1/3

== system ASM_Traffic_MultiCore/Drivetrain/Plant/Drivetrain/Transmission/AutomaticTransmission ==
  Ctrl_Lockup_Clutch[0_1] : Inport
  Gear[] : Inport  Port=2
  n_Engine[rad|s] : Inport  Port=3
  omega_In_Diff[rad|s] : Inport  Port=4
  Reset[0|1] : Inport  Port=5
  Enable_v_Init[0|1] : Inport  Port=6
  Enable : EnablePort  PropagateVarSize=During execution
  ASMSignalCollector : Subsystem
  GEARBOX_AT_RIGID : ASM_VehicleDynamics_lib/Drivetrain/Gearbox/GEARBOX_AT_RIGID  Tag=ASM_SUBCOMPONENT  Map_GearRatio=MDL.Drivetrain.AutomaticTransmission.GearboxATRigid.Map_GearRatio  Const_SyncTime=MDL.Drivetrain.AutomaticTransmission.GearboxATRigid.Const_SyncTime  Const_Inertia_InputGear=MDL.Drivetrain.AutomaticTransmission.GearboxATRigid.Const_Inertia_InputGear  Const_Damping_InputGear=MDL.Drivetrain.AutomaticTransmission.GearboxATRigid.Const_Damping_InputGear  Map_Forward_Efficiency=MDL.Drivetrain.AutomaticTransmission.GearboxATRigid.Map_Forward_Efficiency  Map_Reverse_Efficiency=MDL.Drivetrain.AutomaticTransmission.GearboxATRigid.Map_Reverse_Efficiency  StepSize=SIM.StepSize  ASMProperties=struct('Name','GEARBOX_AT_RIGID','Version','5.0','Library','ASM_VehicleDynamics_lib')  ASMInstanceName=gearbox_at_rigid  ASMInstanceID=1
  Goto Tag Visibility1 : GotoTagVisibility  GotoTag=ASMBUS_AT_LockUpClutch
  Goto Tag Visibility2 : GotoTagVisibility  GotoTag=ASMBUS_AT_Gearbox
  Goto Tag Visibility3 : GotoTagVisibility  GotoTag=ASMBUS_AT_TorqueConverter
  LOCKUP_CLUTCH_RIGID : ASM_VehicleDynamics_lib/Drivetrain/Clutch/LOCKUP_CLUTCH_RIGID  Tag=ASM_SUBCOMPONENT  Const_Torque_Max=MDL.Drivetrain.AutomaticTransmission.LockupClutchRigid.Const_Torque_Max  Map_Trq_Clutch_Red=MDL.Drivetrain.AutomaticTransmission.LockupClutchRigid.Map_Trq_Clutch_Red  Const_Stiffness_Fric_LockupClutch=MDL.Drivetrain.AutomaticTransmission.LockupClutchRigid.Const_Stiffness_Fric_LockupClutch  Const_Damping_Fric_LockupClutch=MDL.Drivetrain.AutomaticTransmission.LockupClutchRigid.Const_Damping_Fric_LockupClutch  StepSize=SIM.StepSize  ASMProperties=struct('Name','LOCKUP_CLUTCH_RIGID','Version','2.0','Library','ASM_VehicleDynamics_lib')  ASMInstanceName=lockup_clutch_rigid  ASMInstanceID=1
  TORQUE_CONVERTER_RIGID : ASM_VehicleDynamics_lib/Drivetrain/Clutch/TORQUE_CONVERTER_RIGID  Tag=ASM_SUBCOMPONENT  Map_Eta_Slip=MDL.Drivetrain.AutomaticTransmission.TorqueConverterRigid.Map_Eta_Slip  Map_Rel_Trq_PumpTurb=MDL.Drivetrain.AutomaticTransmission.TorqueConverterRigid.Map_Rel_Trq_PumpTurb  ASMProperties=struct('Name','TORQUE_CONVERTER_RIGID','Version','2.0','Library','ASM_VehicleDynamics_lib')  ASMInstanceName=torque_converter_rigid  ASMInstanceID=1
  Torque_Summation : Subsystem
  UnitConversion : ASM_Utils_lib/UnitConversion/UnitConversion  Selection=[0_1]_to_%
  avoid_incomplete_trace2source : Subsystem
  avoid_incomplete_trace2source1 : Subsystem
  ASMSignalBus : Outport  VectorParamsAs1DForOutWhenUnconnected=off
  Trq_In_Converter[Nm] : Outport  Port=2  VectorParamsAs1DForOutWhenUnconnected=off
  omega_In_Trm[rad|s] : Outport  Port=3  VectorParamsAs1DForOutWhenUnconnected=off
  Trq_Out_Trm[Nm] : Outport  Port=4  VectorParamsAs1DForOutWhenUnconnected=off
  tag scope: ASMBUS_AT_Gearbox=scoped, ASMBUS_AT_LockUpClutch=scoped, ASMBUS_AT_TorqueConverter=scoped
  wires:
  avoid_incomplete_trace2source1/1(Out1) -> LOCKUP_CLUTCH_RIGID/4
  avoid_incomplete_trace2source/1(Out1) -> GEARBOX_AT_RIGID/3
  omega_In_Diff[rad|s]/1 -> avoid_incomplete_trace2source/1(In1)
  Enable_v_Init[0|1]/1 -> GEARBOX_AT_RIGID/5
  Gear[]/1 -> GEARBOX_AT_RIGID/2
  UnitConversion/1 -> LOCKUP_CLUTCH_RIGID/2
  ASMSignalCollector/1(ASMSignalBus) -> ASMSignalBus/1
  TORQUE_CONVERTER_RIGID/1 -> [ASMBUS_AT_TorqueConverter]
  LOCKUP_CLUTCH_RIGID/1 -> [ASMBUS_AT_LockUpClutch]
  LOCKUP_CLUTCH_RIGID/2 -> Torque_Summation/1(Trq_Fric[Nm])
  Torque_Summation/2(Trq_In_Trm[Nm]) -> GEARBOX_AT_RIGID/1
  Torque_Summation/1(Trq_In_Converter[Nm]) -> Trq_In_Converter[Nm]/1
  TORQUE_CONVERTER_RIGID/3 -> Torque_Summation/3(Trq_Turbine[Nm])
  TORQUE_CONVERTER_RIGID/2 -> Torque_Summation/2(Trq_Pump[Nm])
  GEARBOX_AT_RIGID/3 -> Trq_Out_Trm[Nm]/1
  GEARBOX_AT_RIGID/1 -> [ASMBUS_AT_Gearbox]
  Reset[0|1]/1 -> LOCKUP_CLUTCH_RIGID/3, GEARBOX_AT_RIGID/4
  GEARBOX_AT_RIGID/2 -> TORQUE_CONVERTER_RIGID/2, omega_In_Trm[rad|s]/1, avoid_incomplete_trace2source1/1(In1)
  Ctrl_Lockup_Clutch[0_1]/1 -> UnitConversion/1
  n_Engine[rad|s]/1 -> TORQUE_CONVERTER_RIGID/1, LOCKUP_CLUTCH_RIGID/1

== system ASM_Traffic_MultiCore/Drivetrain/Plant/Drivetrain/Transmission/ManualTransmission ==
  Pos_ClutchPedal[%] : Inport
  Gear[] : Inport  Port=2
  n_Engine[rad|s] : Inport  Port=3
  omega_In_Diff[rad|s] : Inport  Port=4
  Reset[0|1] : Inport  Port=5
  Enable_v_Init[0|1] : Inport  Port=6
  Enable : EnablePort  PropagateVarSize=During execution
  ASMSignalCollector : Subsystem
  CLUTCH_RIGID : ASM_VehicleDynamics_lib/Drivetrain/Clutch/CLUTCH_RIGID  Tag=ASM_SUBCOMPONENT  Const_Torque_Max=MDL.Drivetrain.ManualTransmission.ClutchRigid.Const_Torque_Max  Map_Trq_Clutch_Red=MDL.Drivetrain.ManualTransmission.ClutchRigid.Map_Trq_Clutch_Red  Const_Stiffness_Fric_Clutch=MDL.Drivetrain.ManualTransmission.ClutchRigid.Const_Stiffness_Fric_Clutch  Const_Damping_Fric_Clutch=MDL.Drivetrain.ManualTransmission.ClutchRigid.Const_Damping_Fric_Clutch  StepSize=SIM.StepSize  ASMProperties=struct('Name','CLUTCH_RIGID','Version','2.0','Library','ASM_VehicleDynamics_lib')  ASMInstanceName=clutch_rigid  ASMInstanceID=1
  GEARBOX_MT_RIGID : ASM_VehicleDynamics_lib/Drivetrain/Gearbox/GEARBOX_MT_RIGID  Tag=ASM_SUBCOMPONENT  Map_GearRatio=MDL.Drivetrain.ManualTransmission.GearboxMTRigid.Map_GearRatio  Const_SyncTime=MDL.Drivetrain.ManualTransmission.GearboxMTRigid.Const_SyncTime  Const_Inertia_InputGear=MDL.Drivetrain.ManualTransmission.GearboxMTRigid.Const_Inertia_InputGear  Const_Damping_InputGear=MDL.Drivetrain.ManualTransmission.GearboxMTRigid.Const_Damping_InputGear  Map_Forward_Efficiency=MDL.Drivetrain.ManualTransmission.GearboxMTRigid.Map_Forward_Efficiency  Map_Reverse_Efficiency=MDL.Drivetrain.ManualTransmission.GearboxMTRigid.Map_Reverse_Efficiency  StepSize=SIM.StepSize  ASMProperties=struct('Name','GEARBOX_MT_RIGID','Version','5.0','Library','ASM_VehicleDynamics_lib')  ASMInstanceName=gearbox_mt_rigid  ASMInstanceID=1
  Goto Tag Visibility1 : GotoTagVisibility  GotoTag=ASMBUS_MT_Clutch
  Goto Tag Visibility2 : GotoTagVisibility  GotoTag=ASMBUS_MT_Gearbox
  avoid_incomplete_trace2source : Subsystem
  avoid_incomplete_trace2source1 : Subsystem
  ASMSignalBus : Outport  VectorParamsAs1DForOutWhenUnconnected=off
  Trq_Fric[Nm] : Outport  Port=2  VectorParamsAs1DForOutWhenUnconnected=off
  omega_In_Trm[rad|s] : Outport  Port=3  VectorParamsAs1DForOutWhenUnconnected=off
  Trq_Out_Trm[Nm] : Outport  Port=4  VectorParamsAs1DForOutWhenUnconnected=off
  tag scope: ASMBUS_MT_Clutch=scoped, ASMBUS_MT_Gearbox=scoped
  wires:
  avoid_incomplete_trace2source1/1(Out1) -> GEARBOX_MT_RIGID/3
  omega_In_Diff[rad|s]/1 -> avoid_incomplete_trace2source1/1(In1)
  avoid_incomplete_trace2source/1(Out1) -> CLUTCH_RIGID/4
  Enable_v_Init[0|1]/1 -> GEARBOX_MT_RIGID/5
  ASMSignalCollector/1(ASMSignalBus) -> ASMSignalBus/1
  CLUTCH_RIGID/1 -> [ASMBUS_MT_Clutch]
  GEARBOX_MT_RIGID/1 -> [ASMBUS_MT_Gearbox]
  Reset[0|1]/1 -> CLUTCH_RIGID/3, GEARBOX_MT_RIGID/4
  GEARBOX_MT_RIGID/2 -> avoid_incomplete_trace2source/1(In1), omega_In_Trm[rad|s]/1
  CLUTCH_RIGID/2 -> Trq_Fric[Nm]/1, GEARBOX_MT_RIGID/1
  GEARBOX_MT_RIGID/3 -> Trq_Out_Trm[Nm]/1
  Gear[]/1 -> GEARBOX_MT_RIGID/2
  n_Engine[rad|s]/1 -> CLUTCH_RIGID/1
  Pos_ClutchPedal[%]/1 -> CLUTCH_RIGID/2

== system ASM_Traffic_MultiCore/Drivetrain/Plant/UserInterface/DISP_Plant/ActiveTransmission ==
  ActiveTrm : Inport
  ActiveTransmission : Scope  NumInputPorts=7
      settings: TimeSpan=5  ActiveDisplayYMinimum=0  ActiveDisplayYMaximum=400  DataLoggingMaxPoints=20000  DataLoggingDecimation=10  DataLoggingVariableName=ScopeData47
  Bus Selector : BusSelector  OutputSignals=omega_In_Trm[rad|s],omega_Out_Trm[rad|s],Trq_Out_Trm[Nm],i_Trm[],Inertia_Trm[kgm2],i_unsync_Trm[],Gear[]
  Gear[] : Subsystem
      mask Display: disp('')
  Inertia_Trm[kgm2] : Subsystem
      mask Display: disp('')
  Trq_Out_Trm[Nm] : Subsystem
      mask Display: disp('')
  i_Trm[] : Subsystem
      mask Display: disp('')
  i_unsync_Trm[] : Subsystem
      mask Display: disp('')
  omega_In_Trm[rad|s] : Subsystem
      mask Display: disp('')
  omega_Out_Trm[rad|s] : Subsystem
      mask Display: disp('')
  wires:
  Gear[]/1(Out1) -> ActiveTransmission/7  "Gear[]"
  Bus Selector/7 -> Gear[]/1(In1)  "<Gear[]>"
  i_unsync_Trm[]/1(Out1) -> ActiveTransmission/6  "i_unsync_Trm[]"
  Bus Selector/6 -> i_unsync_Trm[]/1(In1)  "<i_unsync_Trm[]>"
  Inertia_Trm[kgm2]/1(Out1) -> ActiveTransmission/5  "Inertia_Trm[kgm2]"
  Bus Selector/5 -> Inertia_Trm[kgm2]/1(In1)  "<Inertia_Trm[kgm2]>"
  i_Trm[]/1(Out1) -> ActiveTransmission/4  "i_Trm[]"
  Bus Selector/4 -> i_Trm[]/1(In1)  "<i_Trm[]>"
  Trq_Out_Trm[Nm]/1(Out1) -> ActiveTransmission/3  "Trq_Out_Trm[Nm]"
  Bus Selector/3 -> Trq_Out_Trm[Nm]/1(In1)  "<Trq_Out_Trm[Nm]>"
  omega_Out_Trm[rad|s]/1(Out1) -> ActiveTransmission/2  "omega_Out_Trm[rad|s]"
  Bus Selector/2 -> omega_Out_Trm[rad|s]/1(In1)  "<omega_Out_Trm[rad|s]>"
  omega_In_Trm[rad|s]/1(Out1) -> ActiveTransmission/1  "omega_In_Trm[rad|s]"
  Bus Selector/1 -> omega_In_Trm[rad|s]/1(In1)  "<omega_In_Trm[rad|s]>"
  ActiveTrm/1 -> Bus Selector/1

== system ASM_Traffic_MultiCore/Drivetrain/Plant/UserInterface/DISP_Plant/AutomaticTransmission ==
  AutoTrm : Inport
  Bus Selector : BusSelector  OutputSignals=LockUpClutch.Trq_Fric_Clutch[Nm],LockUpClutch.Trq_TorsionSpring_Clutch[Nm],LockUpClutch.omega_Out_ClutchPlate[rad|s],TorqueConverter.Trq_Turbine[Nm],TorqueConverter.Trq_Pump[Nm]
  LookUpClutch : Scope  NumInputPorts=3
      settings: TimeSpan=5  ActiveDisplayYMinimum=-40  ActiveDisplayYMaximum=40  DataLoggingMaxPoints=20000  DataLoggingDecimation=10  DataLoggingVariableName=ScopeData47
  TorqueConverter : Scope  NumInputPorts=2
      settings: TimeSpan=5  ActiveDisplayYMinimum=-40  ActiveDisplayYMaximum=40  DataLoggingMaxPoints=20000  DataLoggingDecimation=10  DataLoggingVariableName=ScopeData65
  Trq_Fric_Clutch[Nm] : Subsystem
      mask Display: disp('')
  Trq_Pump[Nm] : Subsystem
      mask Display: disp('')
  Trq_TorsionSpring_Clutch[Nm] : Subsystem
      mask Display: disp('')
  Trq_Turbine[Nm] : Subsystem
      mask Display: disp('')
  omega_Out_ClutchPlate[rad|s] : Subsystem
      mask Display: disp('')
  wires:
  Bus Selector/5 -> Trq_Pump[Nm]/1(In1)  "<Trq_Pump[Nm]>"
  Bus Selector/4 -> Trq_Turbine[Nm]/1(In1)  "<Trq_Turbine[Nm]>"
  Bus Selector/3 -> omega_Out_ClutchPlate[rad|s]/1(In1)  "<omega_Out_ClutchPlate[rad|s]>"
  Bus Selector/2 -> Trq_TorsionSpring_Clutch[Nm]/1(In1)  "<Trq_TorsionSpring_Clutch[Nm]>"
  Bus Selector/1 -> Trq_Fric_Clutch[Nm]/1(In1)  "<Trq_Fric_Clutch[Nm]>"
  Trq_Pump[Nm]/1(Out1) -> TorqueConverter/2  "Trq_Pump[Nm]"
  Trq_Turbine[Nm]/1(Out1) -> TorqueConverter/1  "Trq_Turbine[Nm]"
  omega_Out_ClutchPlate[rad|s]/1(Out1) -> LookUpClutch/3  "omega_Out_ClutchPlate[rad|s]"
  Trq_TorsionSpring_Clutch[Nm]/1(Out1) -> LookUpClutch/2  "Trq_TorsionSpring_Clutch[Nm]"
  Trq_Fric_Clutch[Nm]/1(Out1) -> LookUpClutch/1  "Trq_Fric_Clutch[Nm]"
  AutoTrm/1 -> Bus Selector/1

== system ASM_Traffic_MultiCore/Drivetrain/Plant/UserInterface/DISP_Plant/EngineSpeed ==
  Crankshaft : Inport
  Starter : Inport  Port=2
  Bus Selector : BusSelector  OutputSignals=n_Engine[rpm]
  Bus Selector1 : BusSelector  OutputSignals=Trq_Starter[Nm]
  EngineSpeed : Scope  NumInputPorts=2
      settings: TimeSpan=5  ActiveDisplayYMinimum=-762.27148  ActiveDisplayYMaximum=6860.44332  DataLoggingMaxPoints=20000  DataLoggingDecimation=10  DataLoggingVariableName=ScopeData47
  Trq_Starter[Nm] : Subsystem
      mask Display: disp('')
  n_Engine[rpm] : Subsystem
      mask Display: disp('')
  wires:
  Starter/1 -> Bus Selector1/1
  Trq_Starter[Nm]/1(Out1) -> EngineSpeed/2  "Trq_Starter[Nm]"
  Bus Selector1/1 -> Trq_Starter[Nm]/1(In1)  "<Trq_Starter[Nm]>"
  n_Engine[rpm]/1(Out1) -> EngineSpeed/1  "n_Engine[rpm]"
  Bus Selector/1 -> n_Engine[rpm]/1(In1)  "<n_Engine[rpm]>"
  Crankshaft/1 -> Bus Selector/1

== system ASM_Traffic_MultiCore/Drivetrain/Plant/UserInterface/DISP_Plant/ManualTransmission ==
  ManTrm : Inport
  Bus Selector : BusSelector  OutputSignals=Clutch.Trq_Fric_Clutch[Nm],Clutch.Trq_TorsionSpring_Clutch[Nm],Clutch.omega_Out_ClutchPlate[rad|s]
  Clutch : Scope  NumInputPorts=3
      settings: TimeSpan=5  ActiveDisplayYMinimum=-40  ActiveDisplayYMaximum=40  DataLoggingMaxPoints=20000  DataLoggingDecimation=10  DataLoggingVariableName=ScopeData47
  Trq_Fric_Clutch[Nm] : Subsystem
      mask Display: disp('')
  Trq_TorsionSpring_Clutch[Nm] : Subsystem
      mask Display: disp('')
  omega_Out_ClutchPlate[rad|s] : Subsystem
      mask Display: disp('')
  wires:
  Bus Selector/3 -> omega_Out_ClutchPlate[rad|s]/1(In1)  "<omega_Out_ClutchPlate[rad|s]>"
  Bus Selector/2 -> Trq_TorsionSpring_Clutch[Nm]/1(In1)  "<Trq_TorsionSpring_Clutch[Nm]>"
  Bus Selector/1 -> Trq_Fric_Clutch[Nm]/1(In1)  "<Trq_Fric_Clutch[Nm]>"
  omega_Out_ClutchPlate[rad|s]/1(Out1) -> Clutch/3  "omega_Out_ClutchPlate[rad|s]"
  Trq_TorsionSpring_Clutch[Nm]/1(Out1) -> Clutch/2  "Trq_TorsionSpring_Clutch[Nm]"
  Trq_Fric_Clutch[Nm]/1(Out1) -> Clutch/1  "Trq_Fric_Clutch[Nm]"
  ManTrm/1 -> Bus Selector/1

== system ASM_Traffic_MultiCore/Drivetrain/Plant/UserInterface/DISP_Plant/Shafts ==
  Shaft_CF : Inport
  Shaft_CR : Inport  Port=2
  Shaft_FL : Inport  Port=3
  Shaft_FR : Inport  Port=4
  Shaft_RL : Inport  Port=5
  Shaft_RR : Inport  Port=6
  Shafts : Scope  NumInputPorts=6
      settings: TimeSpan=5  ActiveDisplayYMinimum=-40  ActiveDisplayYMaximum=40  DataLoggingMaxPoints=20000  DataLoggingDecimation=10  DataLoggingVariableName=ScopeData47
  Trq_CF_Shaft[Nm] : Subsystem
      mask Display: disp('')
  Trq_CR_Shaft[Nm] : Subsystem
      mask Display: disp('')
  Trq_FL_Shaft[Nm] : Subsystem
      mask Display: disp('')
  Trq_FR_Shaft[Nm] : Subsystem
      mask Display: disp('')
  Trq_RL_Shaft[Nm] : Subsystem
      mask Display: disp('')
  Trq_RR_Shaft[Nm] : Subsystem
      mask Display: disp('')
  wires:
  Shaft_RR/1 -> Trq_RR_Shaft[Nm]/1(In1)
  Shaft_RL/1 -> Trq_RL_Shaft[Nm]/1(In1)
  Shaft_FR/1 -> Trq_FR_Shaft[Nm]/1(In1)
  Shaft_FL/1 -> Trq_FL_Shaft[Nm]/1(In1)
  Shaft_CR/1 -> Trq_CR_Shaft[Nm]/1(In1)
  Shaft_CF/1 -> Trq_CF_Shaft[Nm]/1(In1)
  Trq_RR_Shaft[Nm]/1(Out1) -> Shafts/6  "Trq_RR_Shaft[Nm]"
  Trq_RL_Shaft[Nm]/1(Out1) -> Shafts/5  "Trq_RL_Shaft[Nm]"
  Trq_FR_Shaft[Nm]/1(Out1) -> Shafts/4  "Trq_FR_Shaft[Nm]"
  Trq_FL_Shaft[Nm]/1(Out1) -> Shafts/3  "Trq_FL_Shaft[Nm]"
  Trq_CR_Shaft[Nm]/1(Out1) -> Shafts/2  "Trq_CR_Shaft[Nm]"
  Trq_CF_Shaft[Nm]/1(Out1) -> Shafts/1  "Trq_CF_Shaft[Nm]"

== system ASM_Traffic_MultiCore/Drivetrain/SignalInterface/ASMSignalInterface/signal_structure/InfoBlock ==

== system ASM_Traffic_MultiCore/ElectricalSystem/Plant/ElectricalSystemBasic/Battery_HV/ASMSignalCollector ==
  V_Bat[V] : Inport
  SOC_Bat[%] : Inport  Port=2
  T_Bat[degC] : Inport  Port=3
  BusCreator : BusCreator  Inputs=3
  ASMSignalBus : Outport  VectorParamsAs1DForOutWhenUnconnected=off
  wires:
  BusCreator/1 -> ASMSignalBus/1  "Battery_HV"
  V_Bat[V]/1 -> BusCreator/1  "V_Bat[V]"
  SOC_Bat[%]/1 -> BusCreator/2  "SOC_Bat[%]"
  T_Bat[degC]/1 -> BusCreator/3  "T_Bat[degC]"

== system ASM_Traffic_MultiCore/ElectricalSystem/Plant/ElectricalSystemBasic/Battery_LV/ASMSignalCollector ==
  V_Bat[V] : Inport
  SOC_Bat[%] : Inport  Port=2
  T_Bat[degC] : Inport  Port=3
  BusCreator : BusCreator  Inputs=3
  ASMSignalBus : Outport  VectorParamsAs1DForOutWhenUnconnected=off
  wires:
  T_Bat[degC]/1 -> BusCreator/3  "T_Bat[degC]"
  SOC_Bat[%]/1 -> BusCreator/2  "SOC_Bat[%]"
  V_Bat[V]/1 -> BusCreator/1  "V_Bat[V]"
  BusCreator/1 -> ASMSignalBus/1  "Battery_LV"

== system ASM_Traffic_MultiCore/ElectricalSystem/Plant/ElectricalSystemBasic/DCLink/ASMSignalCollector ==
  V_DCLink[V] : Inport
  BusCreator : BusCreator  Inputs=1
  ASMSignalBus : Outport  VectorParamsAs1DForOutWhenUnconnected=off
  wires:
  V_DCLink[V]/1 -> BusCreator/1  "V_DCLink[V]"
  BusCreator/1 -> ASMSignalBus/1  "DCLink"

== system ASM_Traffic_MultiCore/ElectricalSystem/Plant/UserInterface/DISP_Plant/SOC_HV[%] ==
  In1 : Inport
  Gain : Gain
  Out1 : Outport  VectorParamsAs1DForOutWhenUnconnected=off
  wires:
  In1/1 -> Gain/1
  Gain/1 -> Out1/1

== system ASM_Traffic_MultiCore/ElectricalSystem/Plant/UserInterface/DISP_Plant/SOC_LV[%] ==
  In1 : Inport
  Gain : Gain
  Out1 : Outport  VectorParamsAs1DForOutWhenUnconnected=off
  wires:
  Gain/1 -> Out1/1
  In1/1 -> Gain/1

== system ASM_Traffic_MultiCore/ElectricalSystem/Plant/UserInterface/DISP_Plant/T_Bat_HV[degC] ==
  In1 : Inport
  Gain : Gain
  Out1 : Outport  VectorParamsAs1DForOutWhenUnconnected=off
  wires:
  Gain/1 -> Out1/1
  In1/1 -> Gain/1

== system ASM_Traffic_MultiCore/ElectricalSystem/Plant/UserInterface/DISP_Plant/T_Bat_LV[degC] ==
  In1 : Inport
  Gain : Gain
  Out1 : Outport  VectorParamsAs1DForOutWhenUnconnected=off
  wires:
  In1/1 -> Gain/1
  Gain/1 -> Out1/1

== system ASM_Traffic_MultiCore/ElectricalSystem/Plant/UserInterface/DISP_Plant/V_Bat_HV[V] ==
  In1 : Inport
  Gain : Gain
  Out1 : Outport  VectorParamsAs1DForOutWhenUnconnected=off
  wires:
  In1/1 -> Gain/1
  Gain/1 -> Out1/1

== system ASM_Traffic_MultiCore/ElectricalSystem/Plant/UserInterface/DISP_Plant/V_Bat_LV[V] ==
  In1 : Inport
  Gain : Gain
  Out1 : Outport  VectorParamsAs1DForOutWhenUnconnected=off
  wires:
  In1/1 -> Gain/1
  Gain/1 -> Out1/1

== system ASM_Traffic_MultiCore/ElectricalSystem/Plant/UserInterface/DISP_Plant/V_DCLink[V] ==
  In1 : Inport
  Gain : Gain
  Out1 : Outport  VectorParamsAs1DForOutWhenUnconnected=off
  wires:
  Gain/1 -> Out1/1
  In1/1 -> Gain/1

== system ASM_Traffic_MultiCore/ElectricalSystem/SignalInterface/ASMSignalInterface/signal_structure/InfoBlock ==

== system ASM_Traffic_MultiCore/Engine/Control/SoftECU_Engine/SoftECU_Engine/ASMSignalCollector ==
  Bus Creator : BusCreator  Inputs=5
  ASMSignalBus : Outport  VectorParamsAs1DForOutWhenUnconnected=off
  wires:
  [ASMBUS_ESP_FAST_TORQUE_SET] -> Bus Creator/1
  [ASMBUS_SHIFT_TORQUE_SET] -> Bus Creator/2
  Bus Creator/1 -> ASMSignalBus/1  "Control"
  [ASMBUS_ENGINE_OPERATION] -> Bus Creator/5
  [ASMBUS_TORQUE_INTERVENTION] -> Bus Creator/3
  [ASMBUS_IDLE_SPEED_CONTROL] -> Bus Creator/4

== system ASM_Traffic_MultiCore/Engine/Control/SoftECU_Engine/SoftECU_Engine/DisableReset ==
  note: No start request will be sent, if the engine has not been reset
  Reset_VehicleStates[0|1] : Inport
  Sw_CrankShaft_Reset[0Disabled|1Enabled] : Inport  Port=2
  MultiPortSwitch : MultiPortSwitch  DataPortOrder=Zero-based contiguous  Inputs=2  zeroidx=on
  NO_Reset : Constant  Value=0
  Reset[0|1] : Outport  VectorParamsAs1DForOutWhenUnconnected=off
  wires:
  Reset_VehicleStates[0|1]/1 -> MultiPortSwitch/3
  NO_Reset/1 -> MultiPortSwitch/2
  Sw_CrankShaft_Reset[0Disabled|1Enabled]/1 -> MultiPortSwitch/1
  MultiPortSwitch/1 -> Reset[0|1]/1

== system ASM_Traffic_MultiCore/Engine/Control/SoftECU_Engine/SoftECU_Engine/Torque_Intervention_During_Gear_Shift ==
  Factor_Trq_Engine_Red[%] : Inport
  Pos_AccPedal_Driver[%] : Inport  Port=2
  Product : Product
  Saturation[0_100] : Saturate  UpperLimit=100  LowerLimit=0
  UnitConversion : ASM_Utils_lib/UnitConversion/UnitConversion  Selection=%_to_[0_1]
  Pos_AccPedal[%] : Outport  VectorParamsAs1DForOutWhenUnconnected=off
  wires:
  Pos_AccPedal_Driver[%]/1 -> Product/2
  UnitConversion/1 -> Product/1
  Saturation[0_100]/1 -> Pos_AccPedal[%]/1
  Product/1 -> Saturation[0_100]/1
  Factor_Trq_Engine_Red[%]/1 -> UnitConversion/1

== system ASM_Traffic_MultiCore/Engine/Control/SoftECU_Engine/SoftECU_Engine/Vehicle_Topology_Switch ==
  Vehicle_Topology[-2|-1|0|2] : Inport
  Pos_AccPedal[%] : Inport  Port=2
  Enable_Trq_Request_Extern2[0|1] : Inport  Port=3
  Trq_Request_Extern2[Nm] : Inport  Port=4
  Trq_Request_ICE[Nm] : Inport  Port=5
  Compare To Constant : simulink/Logic and Bit Operations/Compare To Constant  relop===  const=2  OutDataTypeStr=boolean
  Constant : Constant
  Constant1 : Constant  Value=0
  Switch : Switch  Criteria=u2 ~= 0  SaturateOnIntegerOverflow=off  InputSameDT=off
  Switch1 : Switch  Criteria=u2 ~= 0  SaturateOnIntegerOverflow=off  InputSameDT=off
  Switch2 : Switch  Criteria=u2 ~= 0  SaturateOnIntegerOverflow=off  InputSameDT=off
  Pos_AccPedal_Driver[%] : Outport  VectorParamsAs1DForOutWhenUnconnected=off
  Enable_Trq_Extern[0|1] : Outport  Port=2  VectorParamsAs1DForOutWhenUnconnected=off
  Trq_Request_Extern[Nm] : Outport  Port=3  VectorParamsAs1DForOutWhenUnconnected=off
  wires:
  Switch/1 -> Enable_Trq_Extern[0|1]/1
  Switch1/1 -> Trq_Request_Extern[Nm]/1
  Vehicle_Topology[-2|-1|0|2]/1 -> Compare To Constant/1
  Constant/1 -> Switch/1
  Compare To Constant/1 -> Switch1/2, Switch/2, Switch2/2
  Trq_Request_ICE[Nm]/1 -> Switch1/1
  Trq_Request_Extern2[Nm]/1 -> Switch1/3
  Enable_Trq_Request_Extern2[0|1]/1 -> Switch/3
  Switch2/1 -> Pos_AccPedal_Driver[%]/1
  Constant1/1 -> Switch2/1
  Pos_AccPedal[%]/1 -> Switch2/3

== system ASM_Traffic_MultiCore/Engine/Control/SoftECU_Engine/SoftECU_Engine/avoid_incomplete_trace2source ==
  In1 : Inport
  DummyGain : Gain
  Out1 : Outport
  wires:
  DummyGain/1 -> Out1/1
  In1/1 -> DummyGain/1

== system ASM_Traffic_MultiCore/Engine/Control/SoftECU_Engine/SoftECU_Engine/avoid_incomplete_trace2source1 ==
  In1 : Inport
  DummyGain : Gain
  Out1 : Outport
  wires:
  DummyGain/1 -> Out1/1
  In1/1 -> DummyGain/1

== system ASM_Traffic_MultiCore/Engine/Control/UserInterface/DISP_Control/Enable_Trq_Request_Extern1[0|1] ==
  In1 : Inport
  Out1 : Outport  VectorParamsAs1DForOutWhenUnconnected=off
  wires:
  In1/1 -> Out1/1

== system ASM_Traffic_MultiCore/Engine/Control/UserInterface/DISP_Control/Enable_Trq_Request_Extern2[0|1] ==
  In1 : Inport
  Out1 : Outport  VectorParamsAs1DForOutWhenUnconnected=off
  wires:
  In1/1 -> Out1/1

== system ASM_Traffic_MultiCore/Engine/Control/UserInterface/DISP_Control/Enable_Trq_Request_Extern3[0|1] ==
  In1 : Inport
  Out1 : Outport  VectorParamsAs1DForOutWhenUnconnected=off
  wires:
  In1/1 -> Out1/1

== system ASM_Traffic_MultiCore/Engine/Control/UserInterface/DISP_Control/Enable_Trq_Request_Fast[0|1] ==
  In1 : Inport
  Out1 : Outport  VectorParamsAs1DForOutWhenUnconnected=off
  wires:
  In1/1 -> Out1/1

== system ASM_Traffic_MultiCore/Engine/Control/UserInterface/DISP_Control/Pos_AccPedal_Request[%] ==
  In1 : Inport
  Out1 : Outport  VectorParamsAs1DForOutWhenUnconnected=off
  wires:
  In1/1 -> Out1/1

== system ASM_Traffic_MultiCore/Engine/Control/UserInterface/DISP_Control/Pos_AccPedal_Request_Driver[%] ==
  In1 : Inport
  Out1 : Outport  VectorParamsAs1DForOutWhenUnconnected=off
  wires:
  In1/1 -> Out1/1

== system ASM_Traffic_MultiCore/Engine/Control/UserInterface/DISP_Control/State_Engine[0|1|2|3|4] ==
  In1 : Inport
  Out1 : Outport  VectorParamsAs1DForOutWhenUnconnected=off
  wires:
  In1/1 -> Out1/1

== system ASM_Traffic_MultiCore/Engine/Control/UserInterface/DISP_Control/Sw_Starter[0|1] ==
  In1 : Inport
  Out1 : Outport  VectorParamsAs1DForOutWhenUnconnected=off
  wires:
  In1/1 -> Out1/1
